simulink model "XBATT01_reference"  (R2025a)
settings: Solver=FixedStepDiscrete  StartTime=0  StopTime=180  FixedStep=0.050000000000000003  RelTol=1e-3
undefined symbols (not defined in the file): ambient_temperature, cooling_fault_fraction, cooling_fault_time, discharge_current, initial_soc, module_parameter_spread
settings Model: Creator=SimuVerity Contributors  LastModifiedBy=SimuVerity Contributors

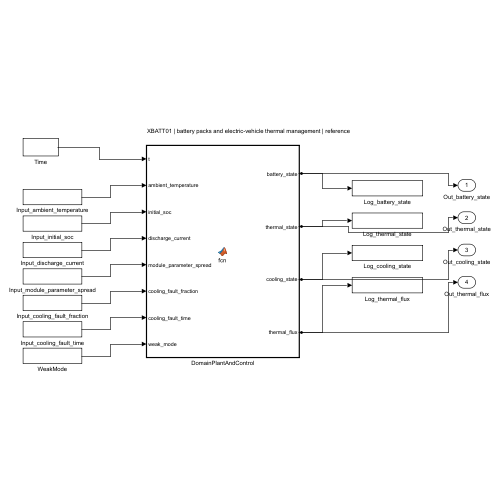
[thumbnail: Simulink's stored preview of the top-level diagram]
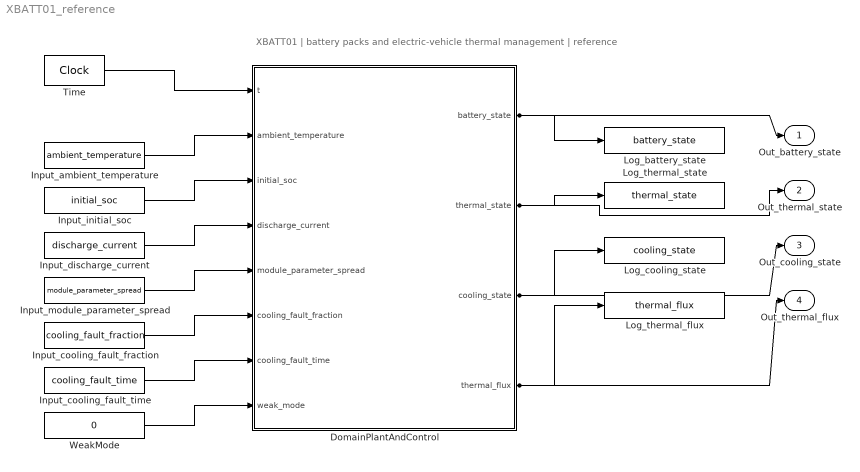
== system XBATT01_reference ==
  note: XBATT01 | battery packs and electric-vehicle thermal management | reference
  DomainPlantAndControl : MATLAB Function  TreatAsAtomicUnit=on
  Input_ambient_temperature : Constant  Value=ambient_temperature
  Input_cooling_fault_fraction : Constant  Value=cooling_fault_fraction
  Input_cooling_fault_time : Constant  Value=cooling_fault_time
  Input_discharge_current : Constant  Value=discharge_current
  Input_initial_soc : Constant  Value=initial_soc
  Input_module_parameter_spread : Constant  Value=module_parameter_spread
  Log_battery_state : ToWorkspace  VariableName=battery_state  SaveFormat=Timeseries  SampleTime=-1
  Log_cooling_state : ToWorkspace  VariableName=cooling_state  SaveFormat=Timeseries  SampleTime=-1
  Log_thermal_flux : ToWorkspace  VariableName=thermal_flux  SaveFormat=Timeseries  SampleTime=-1
  Log_thermal_state : ToWorkspace  VariableName=thermal_state  SaveFormat=Timeseries  SampleTime=-1
  Time : DigitalClock  SampleTime=0.050000000000000003
  WeakMode : Constant  Value=0
  Out_battery_state : Outport
  Out_thermal_state : Outport  Port=2
  Out_cooling_state : Outport  Port=3
  Out_thermal_flux : Outport  Port=4
  wires:
  Time/1 -> DomainPlantAndControl/1(t)
  Input_ambient_temperature/1 -> DomainPlantAndControl/2(ambient_temperature)
  Input_initial_soc/1 -> DomainPlantAndControl/3(initial_soc)
  Input_discharge_current/1 -> DomainPlantAndControl/4(discharge_current)
  Input_module_parameter_spread/1 -> DomainPlantAndControl/5(module_parameter_spread)
  Input_cooling_fault_fraction/1 -> DomainPlantAndControl/6(cooling_fault_fraction)
  Input_cooling_fault_time/1 -> DomainPlantAndControl/7(cooling_fault_time)
  WeakMode/1 -> DomainPlantAndControl/8(weak_mode)
  DomainPlantAndControl/1(battery_state) -> Log_battery_state/1, Out_battery_state/1
  DomainPlantAndControl/2(thermal_state) -> Log_thermal_state/1, Out_thermal_state/1
  DomainPlantAndControl/3(cooling_state) -> Log_cooling_state/1, Out_cooling_state/1
  DomainPlantAndControl/4(thermal_flux) -> Log_thermal_flux/1, Out_thermal_flux/1

== matlab function XBATT01_reference/DomainPlantAndControl ==
  data: t input; battery_state output; ambient_temperature input; initial_soc input; discharge_current input; module_parameter_spread input; cooling_fault_fraction input; cooling_fault_time input; weak_mode input; thermal_state output; cooling_state output; thermal_flux output
function [battery_state,thermal_state,cooling_state,thermal_flux] = fcn(t,ambient_temperature,initial_soc,discharge_current,module_parameter_spread,cooling_fault_fraction,cooling_fault_time,weak_mode)
%#codegen
persistent soc temp pump integ alarmHold faultHold
dt=0.05; capAh=60; Cth=18000; pattern=[-1.0,-0.68,-0.36,-0.12,0.14,0.38,0.70,1.0];
if isempty(soc) || t<0.5*dt
    soc=initial_soc*ones(1,8); temp=ambient_temperature*ones(1,8);
    if weak_mode<.5
        hotDemand=min(max((ambient_temperature-305)/8,0),1); currentDemand=min(max((discharge_current-200)/40,0),1);
        pump=min(max(.25+.20*hotDemand+.25*currentDemand,.12),1);
    else
        pump=.18;
    end
    integ=0; alarmHold=0; faultHold=0;
end
phase=mod(t,36); level=0.94; if phase<12, level=0.82; elseif phase<24, level=1.10; end
current=discharge_current*level;
resistance=.014*(1+module_parameter_spread*pattern).*(1-.004*(temp-298));
ocv=12*(3.30+.78*soc-.03*(1-soc).^2); voltage=ocv-current*resistance;
qGen=current^2*resistance; Tmax=max(temp); spread=max(temp)-min(temp);
target=min(310.5,ambient_temperature+4.2); err=Tmax-target;
if weak_mode<0.5
    integ=min(max(integ+max(err,0)*dt,0),90);
    desired=min(max(.25+.14*max(err,0)+.11*spread+.006*integ,.12),1);
else
    desired=.18;
end
event=double(t>=cooling_fault_time && t<cooling_fault_time+30);
if event>0, faultHold=18; else, faultHold=max(faultHold-dt,0); end
if weak_mode<.5, desired=min(desired+.10*cooling_fault_fraction*double(faultHold>0),1); end
pump=pump+dt*(desired-pump)/1.2;
deliveredFlow=.30*pump*(1-cooling_fault_fraction*event);
pressureDrop=100*(deliveredFlow/.30)^2;
h=245*(1+module_parameter_spread*pattern).*(.22+.58*deliveredFlow/.30);
rawQ=h.*(temp-ambient_temperature); branchCapacity=max(.5*deliveredFlow*4180,1e-6);
scaleL=branchCapacity*(1-exp(-sum(h(1:4))/branchCapacity))/max(sum(h(1:4)),1e-6);
scaleR=branchCapacity*(1-exp(-sum(h(5:8))/branchCapacity))/max(sum(h(5:8)),1e-6);
qCool=[scaleL*rawQ(1:4),scaleR*rawQ(5:8)];
temp=temp+dt*(qGen-qCool)/Cth; soc=max(soc-dt*current/(capAh*3600),0);
qTotal=sum(qCool); leftFlow=max(.5*deliveredFlow,1e-4); rightFlow=leftFlow;
TcoolL=ambient_temperature+sum(qCool(1:4))/(leftFlow*4180);
TcoolR=ambient_temperature+sum(qCool(5:8))/(rightFlow*4180);
auxPower=120*pump^3; bad=(max(temp)>318)||(min(voltage)<36)||(min(soc)<.15);
if bad, alarmHold=8; else, alarmHold=max(alarmHold-dt,0); end
battery_state=[current,sum(voltage),voltage,soc];
thermal_state=[temp,TcoolL,TcoolR];
cooling_state=[pump,deliveredFlow,pressureDrop,auxPower,qTotal,double(alarmHold>0)];
thermal_flux=[qGen,qCool];
end
